simulink model "higher_order_sliding"  (R2016b)
settings: Solver=VariableStepAuto  StartTime=0.0  StopTime=5  RelTol=1e-3
libraries: powerlib_extras x1
settings Model: Creator=Hosein  LastModifiedBy=Hosein

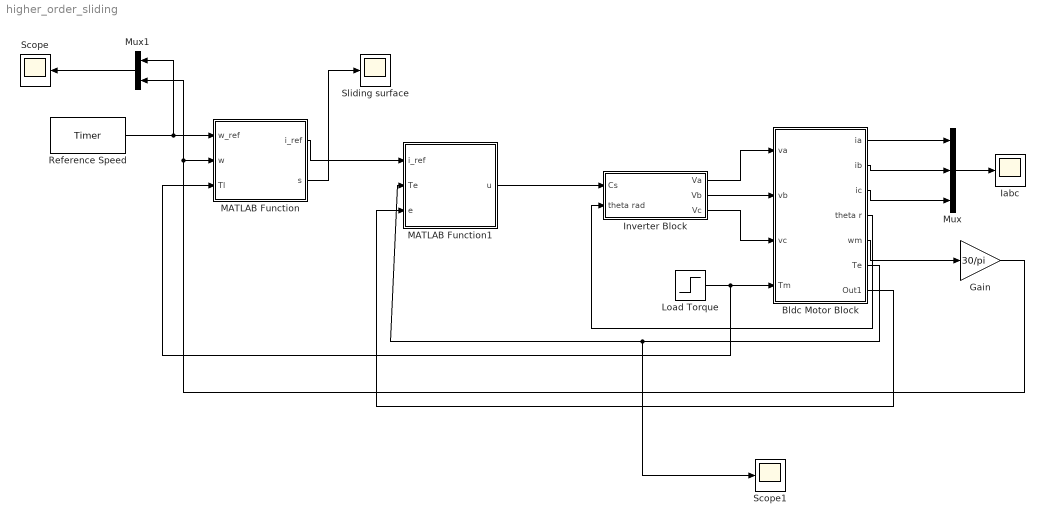
== system higher_order_sliding ==
  Bldc Motor Block : Subsystem
  Gain : Gain  Gain=30/pi
  Iabc : Scope
  Inverter Block : Subsystem
  Load Torque : Step  Time=0.2  After=0.6  SampleTime=0
  MATLAB Function : MATLAB Function  TreatAsAtomicUnit=on
  MATLAB Function1 : MATLAB Function  TreatAsAtomicUnit=on
  Mux : Mux  Inputs=3
  Mux1 : Mux  Inputs=2
  Reference Speed : powerlib_extras/Control  Blocks/Timer  t=[0 0.5 2 4]  e=[2000 1000 3000 500]
  Scope : Scope
  Scope1 : Scope
  Sliding surface : Scope
  wires:
  Inverter Block/2(Vb) -> Bldc Motor Block/2(vb)
  Mux/1 -> Iabc/1
  Inverter Block/1(Va) -> Bldc Motor Block/1(va)
  Bldc Motor Block/1(ia) -> Mux/1
  Bldc Motor Block/2(ib) -> Mux/2
  Bldc Motor Block/3(ic) -> Mux/3
  Inverter Block/3(Vc) -> Bldc Motor Block/3(vc)
  Mux1/1 -> Scope/1
  Load Torque/1 -> MATLAB Function/3(Tl), Bldc Motor Block/4(Tm)
  MATLAB Function/1(i_ref) -> MATLAB Function1/1(i_ref)
  Bldc Motor Block/6(Te) -> Scope1/1, MATLAB Function1/2(Te)
  Bldc Motor Block/5(wm) -> Gain/1
  Gain/1 -> Mux1/2, MATLAB Function/2(w)
  Reference Speed/1 -> Mux1/1, MATLAB Function/1(w_ref)
  MATLAB Function1/1(u) -> Inverter Block/1(Cs)
  Bldc Motor Block/4(theta r) -> Inverter Block/2(theta rad)
  MATLAB Function/2(s) -> Sliding surface/1
  Bldc Motor Block/7(Out1) -> MATLAB Function1/3(e)

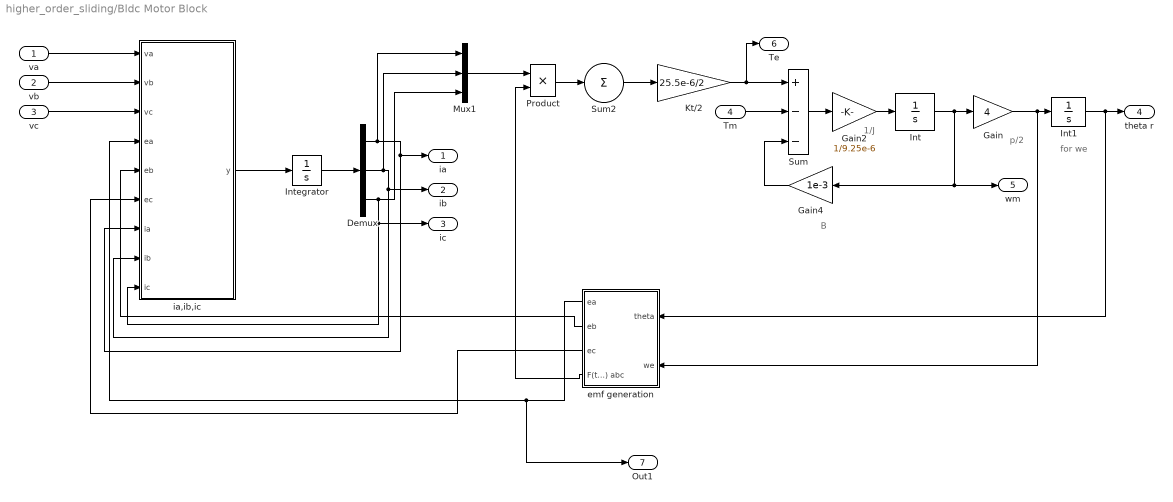
== system higher_order_sliding/Bldc Motor Block ==
  note: 1/J
  note: B
  note: p/2
  note: for we
  va : Inport
  vb : Inport  Port=2
  vc : Inport  Port=3
  Tm : Inport  Port=4
  Demux : Demux  Outputs=3
  Gain : Gain  Gain=4  SaturateOnIntegerOverflow=on  OutDataTypeStr=Inherit: Same as input  ParamDataTypeStr=Inherit: Same as input
  Gain2 : Gain  Gain=1/9.25e-6  SaturateOnIntegerOverflow=on  OutDataTypeStr=Inherit: Same as input  ParamDataTypeStr=Inherit: Same as input
  Gain4 : Gain  Gain=1e-3  SaturateOnIntegerOverflow=on  OutDataTypeStr=Inherit: Same as input  ParamDataTypeStr=Inherit: Same as input
  Int : Integrator
  Int1 : Integrator
  Integrator : Integrator  InitialCondition=0.01
  Kt/2 : Gain  Gain=25.5e-6/2  SaturateOnIntegerOverflow=on  OutDataTypeStr=Inherit: Same as input  ParamDataTypeStr=Inherit: Same as input
  Mux1 : Mux  Inputs=3
  Product : Product  SaturateOnIntegerOverflow=on  OutDataTypeStr=Inherit: Same as first input
  Sum : Sum  Inputs=+--  SaturateOnIntegerOverflow=on  InputSameDT=on  OutDataTypeStr=Inherit: Same as first input
  Sum2 : Sum  Inputs=+  SaturateOnIntegerOverflow=on
  emf generation : Subsystem
  ia,ib,ic : MATLAB Function  TreatAsAtomicUnit=on
  ia : Outport
  ib : Outport  Port=2
  ic : Outport  Port=3
  theta r : Outport  Port=4
  wm : Outport  Port=5
  Te : Outport  Port=6
  Out1 : Outport  Port=7
  wires:
  Sum2/1 -> Kt/2/1
  Product/1 -> Sum2/1
  Mux1/1 -> Product/1
  Int/1 -> Gain/1, Gain4/1, wm/1
  Gain2/1 -> Int/1
  Sum/1 -> Gain2/1
  Gain4/1 -> Sum/3
  Tm/1 -> Sum/2
  Kt/2/1 -> Te/1, Sum/1
  emf generation/4(F(theta) abc) -> Product/2
  Gain/1 -> emf generation/2(we), Int1/1
  Int1/1 -> emf generation/1(theta), theta r/1
  Demux/2 -> Mux1/2, ib/1, ia,ib,ic/8(ib)
  Integrator/1 -> Demux/1
  Demux/3 -> Mux1/3, ia,ib,ic/9(ic), ic/1
  va/1 -> ia,ib,ic/1(va)
  ia,ib,ic/1(y) -> Integrator/1
  vc/1 -> ia,ib,ic/3(vc)
  Demux/1 -> Mux1/1, ia,ib,ic/7(ia), ia/1
  vb/1 -> ia,ib,ic/2(vb)
  emf generation/1(ea) -> Out1/1, ia,ib,ic/4(ea)
  emf generation/2(eb) -> ia,ib,ic/5(eb)
  emf generation/3(ec) -> ia,ib,ic/6(ec)

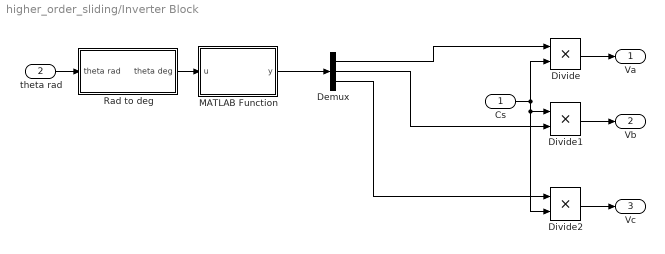
== system higher_order_sliding/Inverter Block ==
  Cs : Inport
  theta rad : Inport  Port=2
  Demux : Demux  Outputs=3
  Divide : Product  Inputs=**
  Divide1 : Product  Inputs=**
  Divide2 : Product  Inputs=**
  MATLAB Function : MATLAB Function  TreatAsAtomicUnit=on
  Rad to deg : Subsystem
  Va : Outport
  Vb : Outport  Port=2
  Vc : Outport  Port=3
  wires:
  theta rad/1 -> Rad to deg/1(theta rad)
  Rad to deg/1(theta deg) -> MATLAB Function/1(u)
  MATLAB Function/1(y) -> Demux/1
  Demux/1 -> Divide/1
  Cs/1 -> Divide/2, Divide2/2, Divide1/1
  Demux/2 -> Divide1/2
  Divide/1 -> Va/1
  Divide1/1 -> Vb/1
  Demux/3 -> Divide2/1
  Divide2/1 -> Vc/1

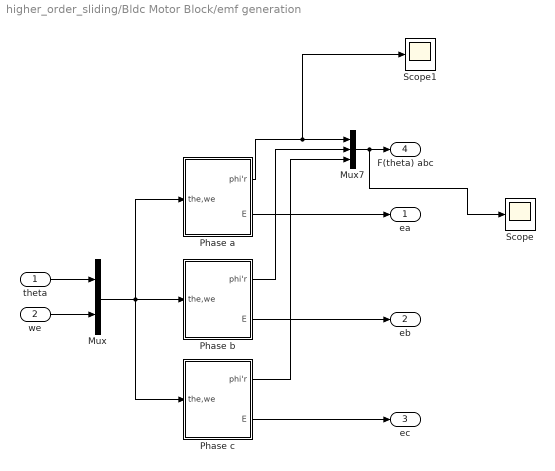
== system higher_order_sliding/Bldc Motor Block/emf generation ==
  theta : Inport
  we : Inport  Port=2
  Mux : Mux  Inputs=2
  Mux7 : Mux  Inputs=3
  Phase a : Subsystem
  Phase b : Subsystem
  Phase c : Subsystem
  Scope : Scope
  Scope1 : Scope
  ea : Outport
  eb : Outport  Port=2
  ec : Outport  Port=3
  F(theta) abc : Outport  Port=4
  wires:
  Mux7/1 -> Scope/1, F(theta) abc/1
  Phase c/1(phi'r) -> Mux7/3
  Phase b/1(phi'r) -> Mux7/2
  Phase a/1(phi'r) -> Scope1/1, Mux7/1
  Mux/1 -> Phase a/1(the,we), Phase b/1(the,we), Phase c/1(the,we)
  Phase a/2(E) -> ea/1
  Phase b/2(E) -> eb/1
  Phase c/2(E) -> ec/1
  theta/1 -> Mux/1
  we/1 -> Mux/2

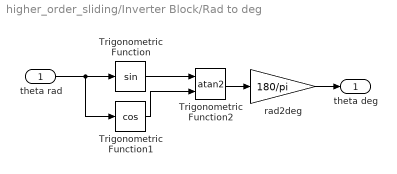
== system higher_order_sliding/Inverter Block/Rad to deg ==
  theta rad : Inport
  Trigonometric Function : Trigonometry
  Trigonometric Function1 : Trigonometry  Operator=cos
  Trigonometric Function2 : Trigonometry  Operator=atan2
  rad2deg : Gain  Gain=180/pi  SaturateOnIntegerOverflow=on  OutDataTypeStr=Inherit: Same as input  ParamDataTypeStr=Inherit: Same as input
  theta deg : Outport
  wires:
  theta rad/1 -> Trigonometric Function/1, Trigonometric Function1/1
  Trigonometric Function/1 -> Trigonometric Function2/1
  Trigonometric Function1/1 -> Trigonometric Function2/2
  Trigonometric Function2/1 -> rad2deg/1
  rad2deg/1 -> theta deg/1

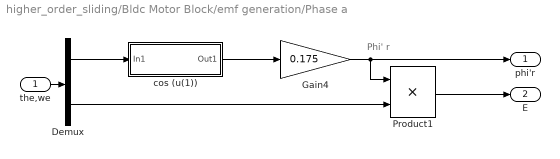
== system higher_order_sliding/Bldc Motor Block/emf generation/Phase a ==
  note: Phi' r
  the,we : Inport
  Demux : Demux  Outputs=2
  Gain4 : Gain  Gain=0.175  SaturateOnIntegerOverflow=on  OutDataTypeStr=Inherit: Same as input  ParamDataTypeStr=Inherit: Same as input
  Product1 : Product  SaturateOnIntegerOverflow=on  OutDataTypeStr=Inherit: Same as first input
  cos (u(1)) : Subsystem
  phi'r : Outport
  E : Outport  Port=2
  wires:
  Gain4/1 -> Product1/1, phi'r/1
  Product1/1 -> E/1
  the,we/1 -> Demux/1
  Demux/2 -> Product1/2
  Demux/1 -> cos (u(1))/1(In1)
  cos (u(1))/1(Out1) -> Gain4/1

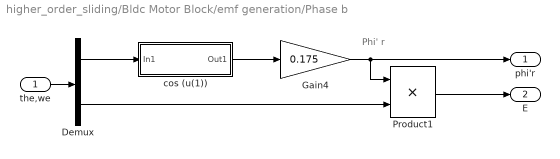
== system higher_order_sliding/Bldc Motor Block/emf generation/Phase b ==
  note: Phi' r
  the,we : Inport
  Demux : Demux  Outputs=2
  Gain4 : Gain  Gain=0.175  SaturateOnIntegerOverflow=on  OutDataTypeStr=Inherit: Same as input  ParamDataTypeStr=Inherit: Same as input
  Product1 : Product  SaturateOnIntegerOverflow=on  OutDataTypeStr=Inherit: Same as first input
  cos (u(1)) : Subsystem
  phi'r : Outport
  E : Outport  Port=2
  wires:
  cos (u(1))/1(Out1) -> Gain4/1
  Demux/1 -> cos (u(1))/1(In1)
  Demux/2 -> Product1/2
  the,we/1 -> Demux/1
  Product1/1 -> E/1
  Gain4/1 -> phi'r/1, Product1/1

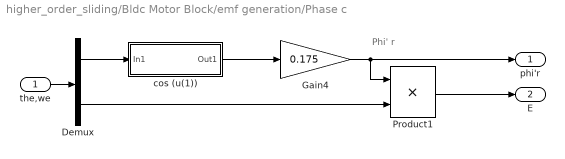
== system higher_order_sliding/Bldc Motor Block/emf generation/Phase c ==
  note: Phi' r
  the,we : Inport
  Demux : Demux  Outputs=2
  Gain4 : Gain  Gain=0.175  SaturateOnIntegerOverflow=on  OutDataTypeStr=Inherit: Same as input  ParamDataTypeStr=Inherit: Same as input
  Product1 : Product  SaturateOnIntegerOverflow=on  OutDataTypeStr=Inherit: Same as first input
  cos (u(1)) : Subsystem
  phi'r : Outport
  E : Outport  Port=2
  wires:
  Gain4/1 -> Product1/1, phi'r/1
  Product1/1 -> E/1
  the,we/1 -> Demux/1
  Demux/2 -> Product1/2
  Demux/1 -> cos (u(1))/1(In1)
  cos (u(1))/1(Out1) -> Gain4/1

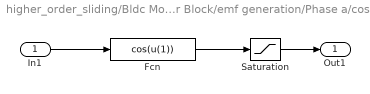
== system higher_order_sliding/Bldc Motor Block/emf generation/Phase a/cos (u(1)) ==
  In1 : Inport
  Fcn : Fcn  Expr=cos(u(1))
  Saturation : Saturate  UpperLimit=0.8  LowerLimit=-0.8
  Out1 : Outport
  wires:
  In1/1 -> Fcn/1
  Fcn/1 -> Saturation/1
  Saturation/1 -> Out1/1

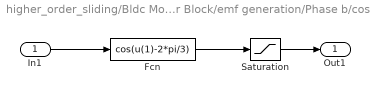
== system higher_order_sliding/Bldc Motor Block/emf generation/Phase b/cos (u(1)) ==
  In1 : Inport
  Fcn : Fcn  Expr=cos(u(1)-2*pi/3)
  Saturation : Saturate  UpperLimit=0.8  LowerLimit=-0.8
  Out1 : Outport
  wires:
  In1/1 -> Fcn/1
  Fcn/1 -> Saturation/1
  Saturation/1 -> Out1/1

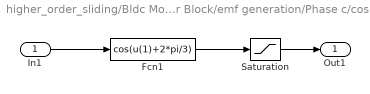
== system higher_order_sliding/Bldc Motor Block/emf generation/Phase c/cos (u(1)) ==
  In1 : Inport
  Fcn1 : Fcn  Expr=cos(u(1)+2*pi/3)
  Saturation : Saturate  UpperLimit=0.8  LowerLimit=-0.8
  Out1 : Outport
  wires:
  In1/1 -> Fcn1/1
  Fcn1/1 -> Saturation/1
  Saturation/1 -> Out1/1

== matlab function higher_order_sliding/Bldc Motor Block/ia,ib,ic ==
  data: va input; y output; vb input; vc input; ea input; eb input; ec input; ia input; ib input; ic input
function y = fcn(va,vb,vc,ea,eb,ec,ia,ib,ic)

Rs = 1.2;        % Ohms, Terminal Resistance phase to phase 
Ls = 0.560e-3;   % Henrys, Terminal Inductance phase to phase 

dia = -(Rs/(Ls))*ia + (1/(Ls))*(va - ea);
dib = -(Rs/(Ls))*ib + (1/(Ls))*(vb - eb);
dic = -(Rs/(Ls))*ic + (1/(Ls))*(vc - ec);

y = [dia;dib;dic];

== matlab function higher_order_sliding/Inverter Block/MATLAB Function ==
  data: u input; y output
function y=emfg(u)
vi=24;
vh=vi/2;
if(u>0)&&(u<=60)
    y=[vi;vh;0];
elseif(u>60)&&(u<=120)
    y=[vh;vi;0];
elseif(u>120)&&(u<=180)
    y=[0;vi;vh];
elseif (u>-180)&&(u<=-120)
    y=[0;vh;vi];
elseif(u>-120)&&(u<=-60)
    y=[vh;0;vi];
else
    y=[vi;0;vh];
end

== matlab function higher_order_sliding/MATLAB Function ==
  data: w_ref input; i_ref output; w input; Tl input; s output
function [i_ref,s] = fcn(w_ref,w,Tl)
Kt = 25.5e-3; 
B=0.001;
J = 92.5e-7;
K=1e4;

s = w-w_ref;
i_ref = J/Kt*((B/J)*w + (1/J)*Tl -K*s);

== matlab function higher_order_sliding/MATLAB Function1 ==
  data: i_ref input; u output; Te input; e input
function u = fcn(i_ref,Te,e)
Kb = 0.0764;
R=1.2;
L = 0.560e-3;
Kt = 25.5e-3;  
K=1e6;

s = Te/Kt - i_ref;

u = L*((R/L)*(Te/Kt) + (1/L)*e -K*s);
